simulink model "cp6_ej4"  (R2026a)
settings: Solver=VariableStepAuto  StopTime=40  MaxStep=0.01
InitFcn:
  | k1 = 4; k2 = 2; T = 3;   % caso 1 (cambiar a k1 = 2; k2 = 4 para el caso 2)
settings Model: Creator=benja  LastModifiedBy=benja

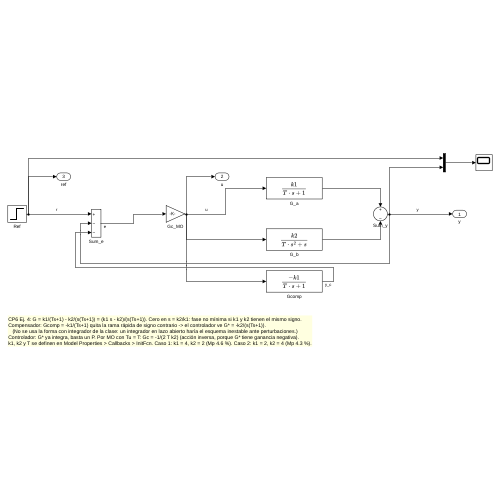
[thumbnail: Simulink's stored preview of the top-level diagram]
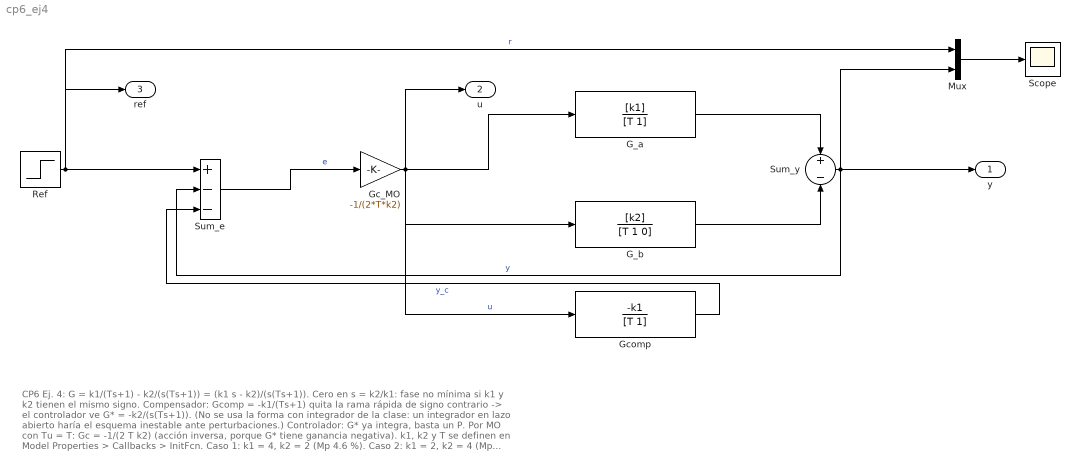
== system cp6_ej4 ==
  note: CP6 Ej. 4: G = k1/(Ts+1) - k2/(s(Ts+1)) = (k1 s - k2)/(s(Ts+1)). Cero en s = k2/k1: fase no mínima si k1 y k2 tienen el mismo signo.
      | Compensador: Gcomp = -k1/(Ts+1) quita la rama rápida de signo contrario -> el controlador ve G* = -k2/(s(Ts+1)).
      |    (No se usa la forma con integrador de la clase: un integrador en lazo abierto haría el esquema inestable ante perturbaciones.)
      | Controlador: G* ya integra, basta un P. Por MO con Tu = T: Gc = -1/(2 T k2) (acción inversa, porque G* tiene ganancia negativa).
      | k1, k2 y T se definen en Model Properties > Callbacks > InitFcn. Caso 1: k1 = 4, k2 = 2 (Mp 4.6 %). Caso 2: k1 = 2, k2 = 4 (Mp 4.3 %).
  G_a : TransferFcn  Numerator=[k1]  Denominator=[T 1]
  G_b : TransferFcn  Numerator=[k2]  Denominator=[T 1 0]
  Gc_MO : Gain  Gain=-1/(2*T*k2)
  Gcomp : TransferFcn  Numerator=-k1  Denominator=[T 1]
  Mux : Mux  Inputs=2
  Ref : Step  SampleTime=0
  Scope : Scope
  Sum_e : Sum  Inputs=+--
  Sum_y : Sum  Inputs=+|-
  y : Outport
  u : Outport  Port=2
  ref : Outport  Port=3
  wires:
  Ref/1 -> Sum_e/1, ref/1, Mux/1  "r"
  Sum_e/1 -> Gc_MO/1  "e"
  Gc_MO/1 -> G_a/1, G_b/1, Gcomp/1, u/1  "u"
  G_a/1 -> Sum_y/1
  G_b/1 -> Sum_y/2
  Sum_y/1 -> y/1, Sum_e/2, Mux/2  "y"
  Gcomp/1 -> Sum_e/3  "y_c"
  Mux/1 -> Scope/1
